simulink model "impmodel"  (R2023a)
settings: Solver=FixedStepDiscrete  StartTime=0.0  StopTime=8  RelTol=1e-3  EnableMultiTasking=on
values from neighbouring files (symbols this model uses):
  availableSpeedModes = 3    [params_f2838.mat]
  inverter_DRV8300 =     [params_f2838.mat]
  PI_params =     [params_f2838.mat]
  pmsm_ECI6360 =     [params_f2838.mat]
  PU_System =     [params_f2838.mat]
  target_f2838 =     [params_f2838.mat]
  Ts = 5e-05    [params_f2838.mat]
  Ts_motor = 2.5e-05    [params_f2838.mat]
  Ts_simulink = 2.5e-05    [params_f2838.mat]
  Ts_speed = 0.0005    [params_f2838.mat]
undefined symbols (not defined in the file or in its folder): Down, GPTRIP1SEL, TZ1, Up
libraries: simulink x35, c2802xlib x11, idelinklib_common x8, procinterlib x8, mcbcontrolslib x8, c280xlib x7, mcbpositiondecoderlib x7, slpidlib x5, svdschedulerlib x4, c2838xlib x2, autolibpmsminterior x1, mcbplantlib x1
(part 1 of 4)
settings Model: ExtModeTrigDuration=8  Creator=baris  LastModifiedBy=baris
settings SolverCC: AutoInsertRateTranBlk=on
settings DataIOCC: LimitDataPoints=on  SaveFormat=Array  SaveOutput=off  SaveTime=off  ReturnWorkspaceOutputs=off
settings OptimizationCC: DefaultUnderspecifiedDataType=single  EnhancedBackFolding=on  PassReuseOutputArgsAs=Individual arguments  MaxStackSize=1024  OptimizeBlockOrder=speed  DifferentSizesBufferReuse=on  DenormalBehavior=FlushToZero  EfficientTunableParamExpr=on
settings DebuggingCC: ReadBeforeWriteMsg=DisableAll  WriteAfterWriteMsg=DisableAll  WriteAfterReadMsg=DisableAll  SignalResolutionControl=TryResolveAllWithWarning  InheritedTsInSrcMsg=none  MultiTaskDSMMsg=none  MultiTaskCondExecSysMsg=none  TasksWithSamePriorityMsg=none  SigSpecEnsureSampleTimeMsg=none  IntegerOverflowMsg=none  ParameterPrecisionLossMsg=none  FcnCallInpInsideContextMsg=warning  UnconnectedInputMsg=warning  UnconnectedOutputMsg=warning  UnconnectedLineMsg=warning  IntegerSaturationMsg=none
settings HardwareCC: ProdBitPerChar=16  ProdBitPerInt=16  ProdBitPerPointer=32  ProdBitPerSizeT=32  ProdBitPerPtrDiffT=32  ProdLargestAtomicInteger=Integer  ProdLargestAtomicFloat=None  ProdWordSize=16  ProdLongLongMode=on  ProdHWDeviceType=Texas Instruments->C2000  HardwareBoardFeatureSet=SoCBlockset
settings ModelReferenceCC: EnableRefExpFcnMdlSchedulingChecks=on  PropagateSignalLabelsOutOfModel=off
settings SFSimCC: MATLABDynamicMemAlloc=off
settings RTWCC: Description=Embedded Coder  SystemTargetFile=ert.tlc  HardwareBoard=TI F2838x  TemplateMakefile=ert_default_tmf  CustomDefine=-DCARPEDIEM_PIN_CORRECTION  Toolchain=Texas Instruments Code Composer Studio - EABI (C2000)
settings CodeAppCC: ForceParamTrailComments=on  IgnoreCustomStorageClasses=off  OperatorAnnotations=on  SimulinkDataObjDesc=on  SFDataObjDesc=on  InsertBlockDesc=on
settings ERTTargetCC: CodeReplacementLibrary=TI C28x  ExtModeTransport=4  ExtModeStaticAlloc=on  ExtModeAutomaticAllocSize=off  ExtModeStaticAllocSize=10000  ExtModeMexFile=ext_xcp  ExtModeIntrfLevel=Level2 - Open
settings ConfigComp: CovEnable=on  RecordCoverage=on  CovModelRefEnable=on

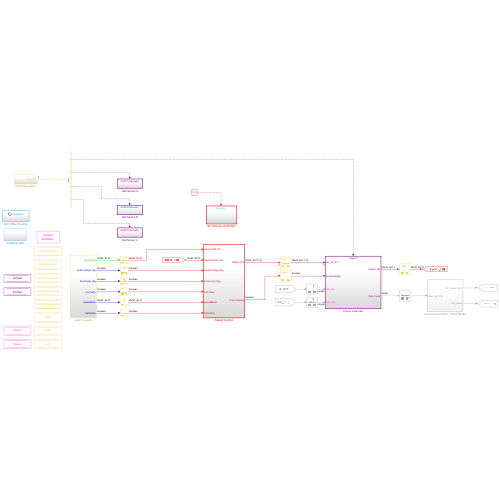
[thumbnail: Simulink's stored preview of the top-level diagram]
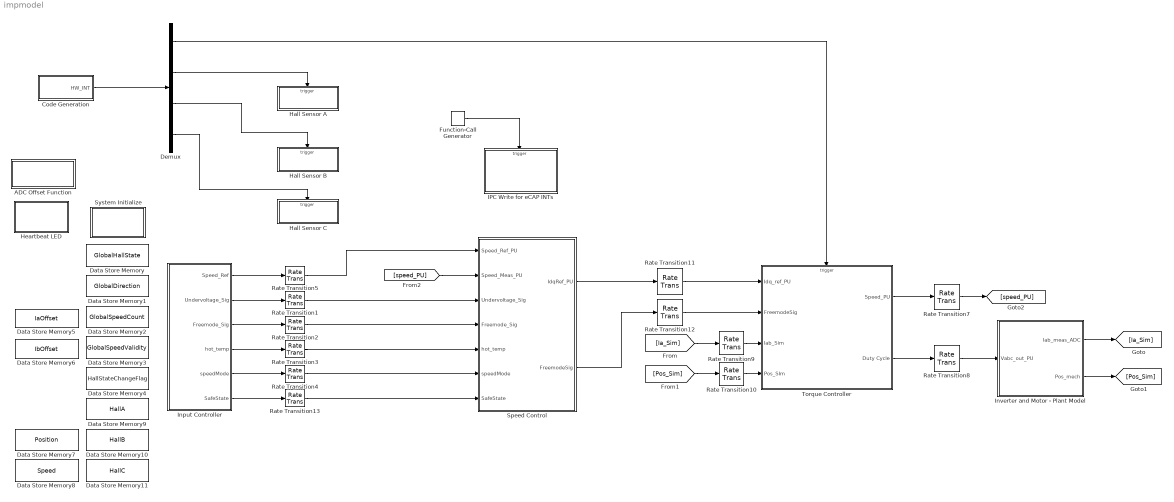
== system impmodel ==
  ADC Offset Function : Subsystem  TreatAsAtomicUnit=on
  Code Generation : Subsystem
  Data Store Memory : DataStoreMemory  DataStoreName=GlobalHallState  WriteAfterWriteMsg=warning  ShowAdditionalParam=off
  Data Store Memory1 : DataStoreMemory  DataStoreName=GlobalDirection  WriteAfterWriteMsg=warning  ShowAdditionalParam=off
  Data Store Memory10 : DataStoreMemory  DataStoreName=HallB  WriteAfterWriteMsg=warning  ShowAdditionalParam=off
  Data Store Memory11 : DataStoreMemory  DataStoreName=HallC  WriteAfterWriteMsg=warning  ShowAdditionalParam=off
  Data Store Memory2 : DataStoreMemory  DataStoreName=GlobalSpeedCount  WriteAfterWriteMsg=warning  ShowAdditionalParam=off
  Data Store Memory3 : DataStoreMemory  DataStoreName=GlobalSpeedValidity  WriteAfterWriteMsg=warning  ShowAdditionalParam=off
  Data Store Memory4 : DataStoreMemory  DataStoreName=HallStateChangeFlag  WriteAfterWriteMsg=warning  ShowAdditionalParam=off
  Data Store Memory5 : DataStoreMemory  DataStoreName=IaOffset  WriteAfterWriteMsg=warning  ShowAdditionalParam=off
  Data Store Memory6 : DataStoreMemory  DataStoreName=IbOffset  WriteAfterWriteMsg=warning  ShowAdditionalParam=off
  Data Store Memory7 : DataStoreMemory  DataStoreName=Position  WriteAfterWriteMsg=warning  ShowAdditionalParam=off
  Data Store Memory8 : DataStoreMemory  DataStoreName=Speed  WriteAfterWriteMsg=warning  ShowAdditionalParam=off
  Data Store Memory9 : DataStoreMemory  DataStoreName=HallA  WriteAfterWriteMsg=warning  ShowAdditionalParam=off
  Demux : Demux
  Function-Call Generator : simulink/Ports & Subsystems/Function-Call Generator  sample_time=-1  numberOfIterations=1  DisallowWideOutput=off
  Hall Sensor A : Subsystem
  Hall Sensor B : Subsystem
  Hall Sensor C : Subsystem
  Heartbeat LED : Subsystem
  IPC Write for eCAP INTs : Subsystem
  Input Controller : Subsystem
  Inverter and Motor - Plant Model : Subsystem
  Rate Transition1 : RateTransition  Deterministic=off  OutPortSampleTime=Ts_speed
  Rate Transition{9..12} (4 alike) : RateTransition  Deterministic=off
  Rate Transition{2..4,13} (4 alike) : RateTransition  Integrity=off  Deterministic=off  OutPortSampleTime=Ts_speed
  Rate Transition5 : RateTransition  Deterministic=off  OutPortSampleTime=Ts_speed
  Rate Transition7 : RateTransition  Deterministic=off  OutPortSampleTime=Ts_speed
  Rate Transition8 : RateTransition  Deterministic=off  OutPortSampleTime=Ts_simulink
  Speed Control : Subsystem  TreatAsAtomicUnit=on  SystemSampleTime=Ts_speed
  System Initialize : Subsystem  mask(System Initialize){ShowInLibBrowser=0}
      mask prompts: ShowInLibBrowser "Simulink:masks:CustCodeMaskParam1_MP"
      settings: CopyFcn=cccopyfcn(gcb)  OpenFcn=ccopenfcn('System Initialize Function')
      mask Help: eval('feval(''rtwprivate'',''rtwhelpview'',''rtw_sys_initialize_block'')');
      mask DialogControl ShowInLibBrowser Prompt: Mask Parameter 1:
      mask Display: disp('System\nInitialize');
  Torque Controller : Subsystem
  wires:
  Code Generation/1(HW_INT) -> Demux/1
  Demux/1 -> Torque Controller/Trigger
  Rate Transition5/1 -> Speed Control/1(Speed_Ref_PU)
  Torque Controller/1(Speed_PU) -> Rate Transition7/1
  [speed_PU] -> Speed Control/2(Speed_Meas_PU)
  Input Controller/1(Speed_Ref) -> Rate Transition5/1
  Input Controller/2(Undervoltage_Sig) -> Rate Transition1/1
  Input Controller/3(Freemode_Sig) -> Rate Transition2/1
  Input Controller/4(hot_temp) -> Rate Transition3/1
  Input Controller/5(speedMode) -> Rate Transition4/1
  Rate Transition1/1 -> Speed Control/3(Undervoltage_Sig)
  Rate Transition2/1 -> Speed Control/4(Freemode_Sig)
  Rate Transition3/1 -> Speed Control/5(hot_temp)
  Rate Transition4/1 -> Speed Control/6(speedMode)
  Inverter and Motor - Plant Model/1(Iab_meas_ADC) -> [Ia_Sim]
  Inverter and Motor - Plant Model/2(Pos_mech) -> [Pos_Sim]
  Torque Controller/2(Duty Cycle) -> Rate Transition8/1
  Rate Transition8/1 -> Inverter and Motor - Plant Model/1(Vabc_out_PU)
  Rate Transition10/1 -> Torque Controller/4(Pos_SIm)
  [Pos_Sim] -> Rate Transition10/1
  [Ia_Sim] -> Rate Transition9/1
  Rate Transition9/1 -> Torque Controller/3(Iab_Sim)
  Speed Control/1(IdqRef_PU) -> Rate Transition11/1
  Speed Control/2(FreemodeSig) -> Rate Transition12/1
  Rate Transition11/1 -> Torque Controller/1(Idq_ref_PU)
  Rate Transition12/1 -> Torque Controller/2(FreemodeSig)
  Rate Transition7/1 -> [speed_PU]
  Input Controller/6(SafeState) -> Rate Transition13/1
  Rate Transition13/1 -> Speed Control/7(SafeState)
  Demux/2 -> Hall Sensor A/Trigger
  Demux/3 -> Hall Sensor B/Trigger
  Demux/4 -> Hall Sensor C/Trigger
  Function-Call Generator/1 -> IPC Write for eCAP INTs/Trigger

== system impmodel/ADC Offset Function ==
  "Calculate ADC Offset " : Subsystem  Priority=1001  TreatAsAtomicUnit=on
  Constant : Constant  Value=inverter_DRV8300.ADCOffsetCalibEnable
  Default ADC Offset : Subsystem  Priority=1001  TreatAsAtomicUnit=on
  Event Listener : EventListener  DisableCoverage=on  EventName=reset
  NOT : Logic  Operator=NOT  IconShape=distinctive  AllPortsSameDT=off  OutDataTypeStr=boolean
  wires:
  Constant/1 -> NOT/1, "Calculate ADC Offset "/Enable
  NOT/1 -> Default ADC Offset/Enable

== system impmodel/Code Generation ==
  CodeGeneration : Subsystem
  Simulation : Subsystem
  Variant Source : VariantSource  VariantControlMode=sim codegen switching  OutputFunctionCall=on
  HW_INT : Outport
  wires:
  Variant Source/1 -> HW_INT/1
  CodeGeneration/1(HW_INT) -> Variant Source/1
  Simulation/1(HW_INT) -> Variant Source/2

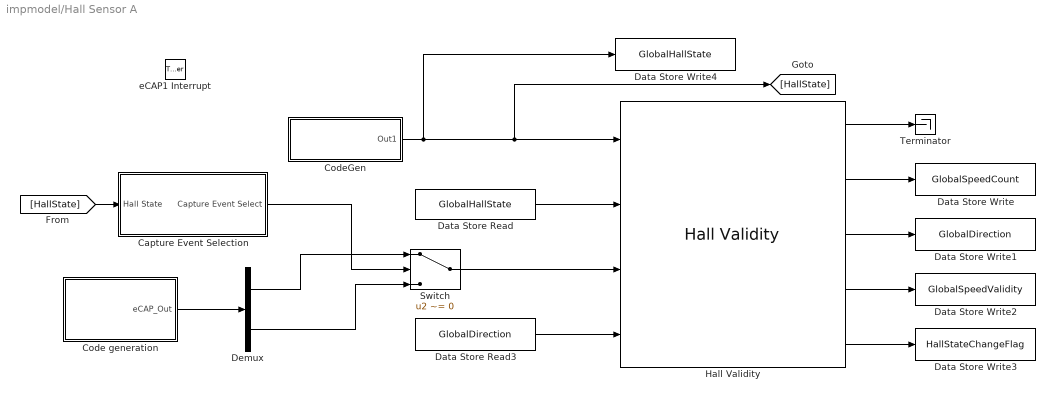
== system impmodel/Hall Sensor A ==
  eCAP1 Interrupt : TriggerPort  TriggerType=function-call  VariantControl=(inherit)  PortDimensions=1
  Capture Event Selection : Subsystem
  Code generation : Subsystem
  CodeGen : Subsystem
  Data Store Read : DataStoreRead  DataStoreName=GlobalHallState  IndexOptions=Index vector (dialog)  Indices=1  OutputSizes=1
  Data Store Read3 : DataStoreRead  DataStoreName=GlobalDirection  IndexOptions=Index vector (dialog)  Indices=1  OutputSizes=1
  Data Store Write : DataStoreWrite  DataStoreName=GlobalSpeedCount  IndexOptions=Index vector (dialog)  Indices=1  OutputSizes=1
  Data Store Write1 : DataStoreWrite  DataStoreName=GlobalDirection  IndexOptions=Index vector (dialog)  Indices=1  OutputSizes=1
  Data Store Write2 : DataStoreWrite  DataStoreName=GlobalSpeedValidity  IndexOptions=Index vector (dialog)  Indices=1  OutputSizes=1
  Data Store Write3 : DataStoreWrite  DataStoreName=HallStateChangeFlag  IndexOptions=Index vector (dialog)  Indices=1  OutputSizes=1
  Data Store Write4 : DataStoreWrite  DataStoreName=GlobalHallState  IndexOptions=Index vector (dialog)  Indices=1  OutputSizes=1
  Demux : Demux  Outputs=2
  Hall Validity : mcbpositiondecoderlib/Hall Validity  hallSequence=ABC  sequence=[5,4,6,2,3,1]  CounterSize=32 bits
      settings: LibrarySourceBlock=mcblib/Sensor Decoders/Hall Validity
  Switch : Switch  Criteria=u2 ~= 0  SaturateOnIntegerOverflow=off  InputSameDT=off
  Terminator : Terminator
  wires:
  Hall Validity/4 -> Data Store Write2/1
  Hall Validity/1 -> Terminator/1
  Hall Validity/5 -> Data Store Write3/1
  Data Store Read3/1 -> Hall Validity/4
  CodeGen/1(Out1) -> Hall Validity/1, [HallState], Data Store Write4/1
  Hall Validity/2 -> Data Store Write/1
  Hall Validity/3 -> Data Store Write1/1
  [HallState] -> Capture Event Selection/1(Hall State)
  Switch/1 -> Hall Validity/3
  Capture Event Selection/1(Capture Event Select) -> Switch/2
  Code generation/1(eCAP_Out) -> Demux/1
  Data Store Read/1 -> Hall Validity/2
  Demux/1 -> Switch/1
  Demux/2 -> Switch/3

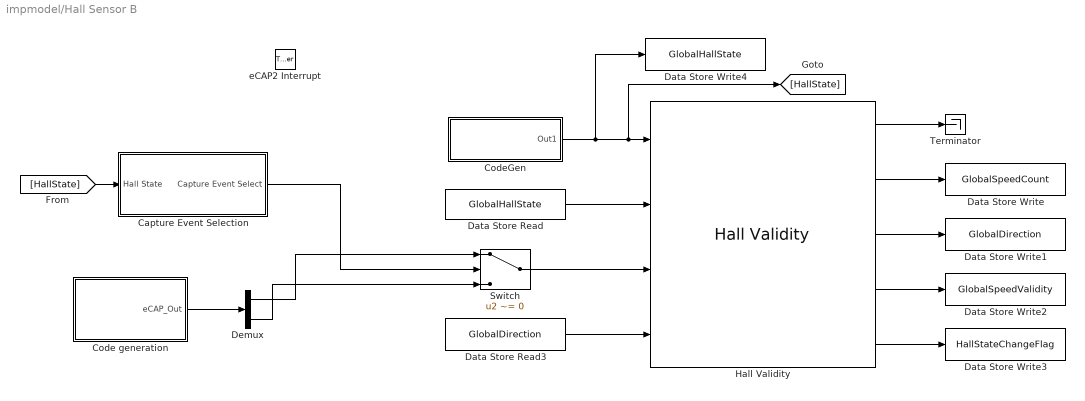
== system impmodel/Hall Sensor B ==
  eCAP2 Interrupt : TriggerPort  TriggerType=function-call  VariantControl=(inherit)  PortDimensions=1
  Capture Event Selection : Subsystem
  Code generation : Subsystem
  CodeGen : Subsystem
  Data Store Read : DataStoreRead  DataStoreName=GlobalHallState  IndexOptions=Index vector (dialog)  Indices=1  OutputSizes=1
  Data Store Read3 : DataStoreRead  DataStoreName=GlobalDirection  IndexOptions=Index vector (dialog)  Indices=1  OutputSizes=1
  Data Store Write : DataStoreWrite  DataStoreName=GlobalSpeedCount  IndexOptions=Index vector (dialog)  Indices=1  OutputSizes=1
  Data Store Write1 : DataStoreWrite  DataStoreName=GlobalDirection  IndexOptions=Index vector (dialog)  Indices=1  OutputSizes=1
  Data Store Write2 : DataStoreWrite  DataStoreName=GlobalSpeedValidity  IndexOptions=Index vector (dialog)  Indices=1  OutputSizes=1
  Data Store Write3 : DataStoreWrite  DataStoreName=HallStateChangeFlag  IndexOptions=Index vector (dialog)  Indices=1  OutputSizes=1
  Data Store Write4 : DataStoreWrite  DataStoreName=GlobalHallState  IndexOptions=Index vector (dialog)  Indices=1  OutputSizes=1
  Demux : Demux  Outputs=2
  Hall Validity : mcbpositiondecoderlib/Hall Validity  hallSequence=ABC  sequence=[5,4,6,2,3,1]  CounterSize=32 bits
      settings: LibrarySourceBlock=mcblib/Sensor Decoders/Hall Validity
  Switch : Switch  Criteria=u2 ~= 0  SaturateOnIntegerOverflow=off  InputSameDT=off
  Terminator : Terminator
  wires:
  Hall Validity/3 -> Data Store Write1/1
  Hall Validity/2 -> Data Store Write/1
  CodeGen/1(Out1) -> [HallState], Hall Validity/1, Data Store Write4/1
  Data Store Read3/1 -> Hall Validity/4
  Hall Validity/5 -> Data Store Write3/1
  Hall Validity/1 -> Terminator/1
  Hall Validity/4 -> Data Store Write2/1
  Capture Event Selection/1(Capture Event Select) -> Switch/2
  [HallState] -> Capture Event Selection/1(Hall State)
  Code generation/1(eCAP_Out) -> Demux/1
  Demux/1 -> Switch/1
  Demux/2 -> Switch/3
  Switch/1 -> Hall Validity/3
  Data Store Read/1 -> Hall Validity/2

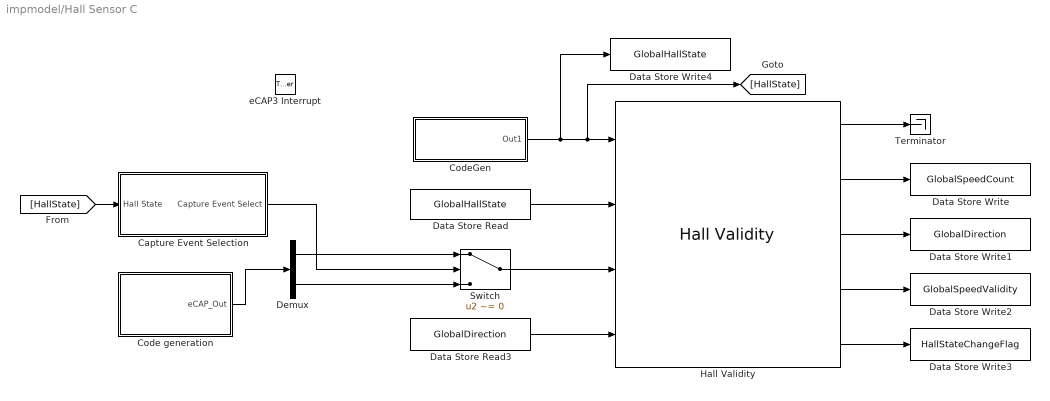
== system impmodel/Hall Sensor C ==
  eCAP3 Interrupt : TriggerPort  TriggerType=function-call  VariantControl=(inherit)  PortDimensions=1
  Capture Event Selection : Subsystem
  Code generation : Subsystem
  CodeGen : Subsystem
  Data Store Read : DataStoreRead  DataStoreName=GlobalHallState  IndexOptions=Index vector (dialog)  Indices=1  OutputSizes=1
  Data Store Read3 : DataStoreRead  DataStoreName=GlobalDirection  IndexOptions=Index vector (dialog)  Indices=1  OutputSizes=1
  Data Store Write : DataStoreWrite  DataStoreName=GlobalSpeedCount  IndexOptions=Index vector (dialog)  Indices=1  OutputSizes=1
  Data Store Write1 : DataStoreWrite  DataStoreName=GlobalDirection  IndexOptions=Index vector (dialog)  Indices=1  OutputSizes=1
  Data Store Write2 : DataStoreWrite  DataStoreName=GlobalSpeedValidity  IndexOptions=Index vector (dialog)  Indices=1  OutputSizes=1
  Data Store Write3 : DataStoreWrite  DataStoreName=HallStateChangeFlag  IndexOptions=Index vector (dialog)  Indices=1  OutputSizes=1
  Data Store Write4 : DataStoreWrite  DataStoreName=GlobalHallState  IndexOptions=Index vector (dialog)  Indices=1  OutputSizes=1
  Demux : Demux  Outputs=2
  Hall Validity : mcbpositiondecoderlib/Hall Validity  hallSequence=ABC  sequence=[5,4,6,2,3,1]  CounterSize=32 bits
      settings: LibrarySourceBlock=mcblib/Sensor Decoders/Hall Validity
  Switch : Switch  Criteria=u2 ~= 0  SaturateOnIntegerOverflow=off  InputSameDT=off
  Terminator : Terminator
  wires:
  Hall Validity/4 -> Data Store Write2/1
  Hall Validity/1 -> Terminator/1
  Hall Validity/5 -> Data Store Write3/1
  Data Store Read3/1 -> Hall Validity/4
  CodeGen/1(Out1) -> Data Store Write4/1, [HallState], Hall Validity/1
  Hall Validity/2 -> Data Store Write/1
  Hall Validity/3 -> Data Store Write1/1
  [HallState] -> Capture Event Selection/1(Hall State)
  Switch/1 -> Hall Validity/3
  Code generation/1(eCAP_Out) -> Demux/1
  Demux/1 -> Switch/1
  Demux/2 -> Switch/3
  Capture Event Selection/1(Capture Event Select) -> Switch/2
  Data Store Read/1 -> Hall Validity/2

== system impmodel/Heartbeat LED ==
  Constant : Constant  SampleTime=0.5
  Digital Output : c2838xlib/Digital Output  GPIO_Number=GPIO56~GPIO63  GPIO_Bit0=on  GPIO_BIT0_Toggle=on  GPIO_Bit1=off  GPIO_BIT1_Toggle=off  GPIO_Bit2=off  GPIO_BIT2_Toggle=off  GPIO_Bit3=off  GPIO_BIT3_Toggle=off  GPIO_Bit4=off  GPIO_BIT4_Toggle=off  GPIO_Bit5=off  GPIO_BIT5_Toggle=off  GPIO_Bit6=off  GPIO_BIT6_Toggle=off  GPIO_Bit7=off  GPIO_BIT7_Toggle=off
  wires:
  Constant/1 -> Digital Output/1

== system impmodel/IPC Write for eCAP INTs ==
  function : TriggerPort  TriggerType=function-call  VariantControl=(inherit)
  Data Store Read2 : DataStoreRead  DataStoreName=GlobalHallState  IndexOptions=Index vector (dialog)  Indices=1  OutputSizes=1
  Data Store Read3 : DataStoreRead  DataStoreName=HallA  IndexOptions=Index vector (dialog)  Indices=1  OutputSizes=1
  Data Store Read4 : DataStoreRead  DataStoreName=HallB  IndexOptions=Index vector (dialog)  Indices=1  OutputSizes=1
  Data Store Read5 : DataStoreRead  DataStoreName=HallC  IndexOptions=Index vector (dialog)  Indices=1  OutputSizes=1
  Memory{2..5} (4 alike) : Memory  InheritSampleTime=on
  TCP_HallA : Subsystem
  TCP_HallB : Subsystem
  TCP_HallC : Subsystem
  TCP_HallState : Subsystem
  wires:
  Data Store Read2/1 -> Memory2/1
  Data Store Read3/1 -> Memory3/1
  Data Store Read4/1 -> Memory4/1
  Data Store Read5/1 -> Memory5/1
  Memory2/1 -> TCP_HallState/1(" ")
  Memory3/1 -> TCP_HallA/1(" ")
  Memory4/1 -> TCP_HallB/1(" ")
  Memory5/1 -> TCP_HallC/1(" ")

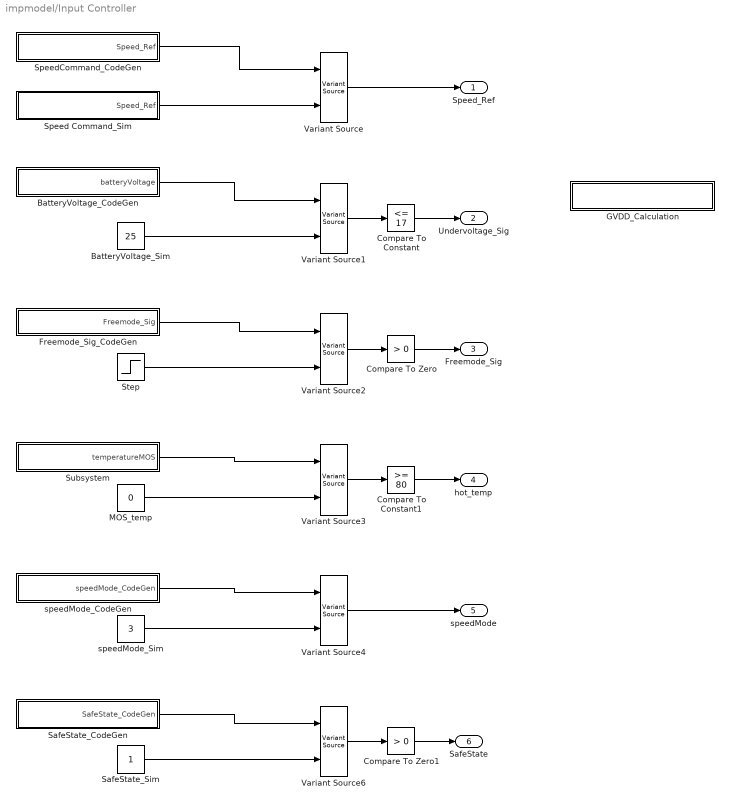
== system impmodel/Input Controller ==
  BatteryVoltage_CodeGen : Subsystem
  BatteryVoltage_Sim : Constant  Value=25  OutDataTypeStr=uint16  SampleTime=0.2
  Compare To Constant : simulink/Logic and Bit Operations/Compare To Constant  relop=<=  const=17  OutDataTypeStr=boolean
  Compare To Constant1 : simulink/Logic and Bit Operations/Compare To Constant  relop=>=  const=80  OutDataTypeStr=boolean
  Compare To Zero : simulink/Logic and Bit Operations/Compare To Zero  relop=>  OutDataTypeStr=boolean
  Compare To Zero1 : simulink/Logic and Bit Operations/Compare To Zero  relop=>  OutDataTypeStr=boolean
  Freemode_Sig_CodeGen : Subsystem
  GVDD_Calculation : Subsystem
  MOS_temp : Constant  Value=0  OutDataTypeStr=uint16  SampleTime=0.2
  SafeState_CodeGen : Subsystem
  SafeState_Sim : Constant  OutDataTypeStr=uint8  SampleTime=0.2
  Speed Command_Sim : Subsystem
  SpeedCommand_CodeGen : Subsystem
  Step : Step  Time=10  After=0  SampleTime=0.2
  Subsystem : Subsystem
  Variant Source{,1..4,6} (6 alike) : VariantSource  VariantControlMode=sim codegen switching
  speedMode_CodeGen : Subsystem
  speedMode_Sim : Constant  Value=3  OutDataTypeStr=uint16  SampleTime=0.2
  Speed_Ref : Outport
  Undervoltage_Sig : Outport  Port=2
  Freemode_Sig : Outport  Port=3
  hot_temp : Outport  Port=4
  speedMode : Outport  Port=5
  SafeState : Outport  Port=6
  wires:
  Variant Source/1 -> Speed_Ref/1
  SpeedCommand_CodeGen/1(Speed_Ref) -> Variant Source/1
  Speed Command_Sim/1(Speed_Ref) -> Variant Source/2
  Variant Source1/1 -> Compare To Constant/1
  BatteryVoltage_CodeGen/1(batteryVoltage) -> Variant Source1/1
  BatteryVoltage_Sim/1 -> Variant Source1/2
  Compare To Constant/1 -> Undervoltage_Sig/1
  Variant Source2/1 -> Compare To Zero/1
  Step/1 -> Variant Source2/2
  Freemode_Sig_CodeGen/1(Freemode_Sig) -> Variant Source2/1
  Subsystem/1(temperatureMOS) -> Variant Source3/1
  MOS_temp/1 -> Variant Source3/2
  Variant Source3/1 -> Compare To Constant1/1
  Compare To Constant1/1 -> hot_temp/1
  Variant Source4/1 -> speedMode/1
  speedMode_Sim/1 -> Variant Source4/2
  speedMode_CodeGen/1(speedMode_CodeGen) -> Variant Source4/1
  Compare To Zero/1 -> Freemode_Sig/1
  Variant Source6/1 -> Compare To Zero1/1
  SafeState_Sim/1 -> Variant Source6/2
  SafeState_CodeGen/1(SafeState_CodeGen) -> Variant Source6/1
  Compare To Zero1/1 -> SafeState/1

== system impmodel/Inverter and Motor - Plant Model ==
  Vabc_out_PU : Inport
  Codegeneration : Subsystem
  Simulation : Subsystem
  Variant Sink : VariantSink  VariantControlMode=sim codegen switching
  Variant Source : VariantSource  VariantControlMode=sim codegen switching
  Variant Source1 : VariantSource  VariantControlMode=sim codegen switching
  Iab_meas_ADC : Outport  VectorParamsAs1DForOutWhenUnconnected=off
  Pos_mech : Outport  Port=2  VectorParamsAs1DForOutWhenUnconnected=off
  wires:
  Codegeneration/2(Pos_fb_Sim) -> Variant Source1/1
  Codegeneration/1(Iab_fb_Sim) -> Variant Source/1
  Variant Source1/1 -> Pos_mech/1
  Variant Sink/1 -> Codegeneration/1(Duty_Cycles)
  Variant Source/1 -> Iab_meas_ADC/1
  Simulation/1(Iab_fb_Sim) -> Variant Source/2
  Variant Sink/2 -> Simulation/1(Duty_Cycles)
  Simulation/2(Pos_fb_Sim) -> Variant Source1/2
  Vabc_out_PU/1 -> Variant Sink/1

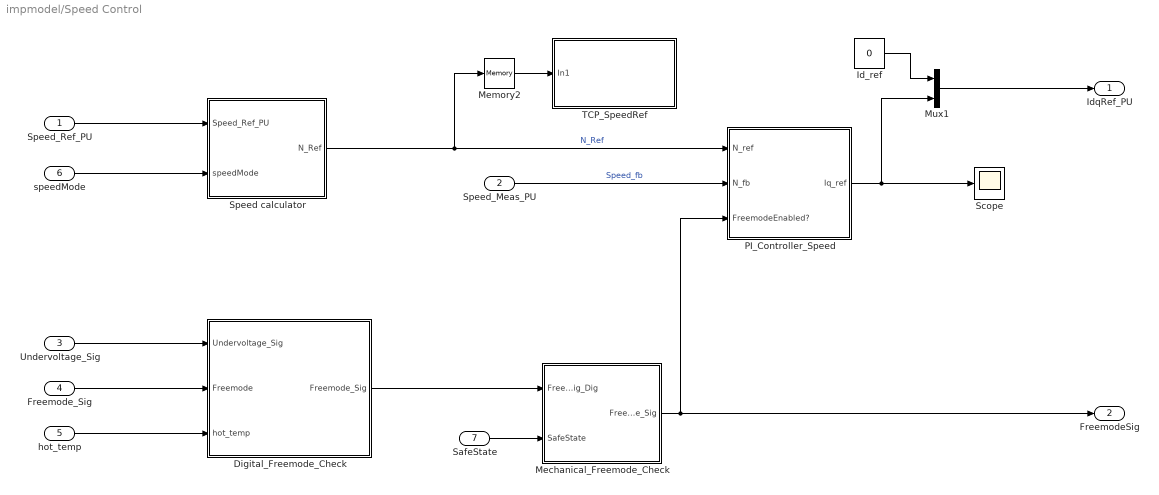
== system impmodel/Speed Control ==
  Speed_Ref_PU : Inport
  Speed_Meas_PU : Inport  Port=2
  Undervoltage_Sig : Inport  Port=3
  Freemode_Sig : Inport  Port=4
  hot_temp : Inport  Port=5
  speedMode : Inport  Port=6
  SafeState : Inport  Port=7
  Digital_Freemode_Check : Subsystem  TreatAsAtomicUnit=on
  Id_ref : Constant  Value=0  OutDataTypeStr=fixdt(1,32,17)  SampleTime=Ts_speed
  Mechanical_Freemode_Check : Subsystem
  Memory2 : Memory  InheritSampleTime=on
  Mux1 : Mux  Inputs=2
  PI_Controller_Speed : Subsystem  TreatAsAtomicUnit=on  SystemSampleTime=Ts_speed
  Scope : Scope
  Speed calculator : Subsystem
  TCP_SpeedRef : Subsystem
  IdqRef_PU : Outport  VectorParamsAs1DForOutWhenUnconnected=off
  FreemodeSig : Outport  Port=2  VectorParamsAs1DForOutWhenUnconnected=off
  wires:
  Id_ref/1 -> Mux1/1
  speedMode/1 -> Speed calculator/2(speedMode)
  Freemode_Sig/1 -> Digital_Freemode_Check/2(Freemode)
  Undervoltage_Sig/1 -> Digital_Freemode_Check/1(Undervoltage_Sig)
  hot_temp/1 -> Digital_Freemode_Check/3(hot_temp)
  Speed_Meas_PU/1 -> PI_Controller_Speed/2(N_fb)  "Speed_fb"
  Mux1/1 -> IdqRef_PU/1
  Speed calculator/1(N_Ref) -> Memory2/1, PI_Controller_Speed/1(N_ref)  "N_Ref"
  Speed_Ref_PU/1 -> Speed calculator/1(Speed_Ref_PU)
  SafeState/1 -> Mechanical_Freemode_Check/2(SafeState)
  PI_Controller_Speed/1(Iq_ref) -> Scope/1, Mux1/2
  Digital_Freemode_Check/1("Freemode_Sig  ") -> Mechanical_Freemode_Check/1(Freemode_Sig_Dig)
  Mechanical_Freemode_Check/1(Freemode_Sig) -> PI_Controller_Speed/3("  FreemodeEnabled?"), FreemodeSig/1
  Memory2/1 -> TCP_SpeedRef/1(In1)

== system impmodel/System Initialize ==

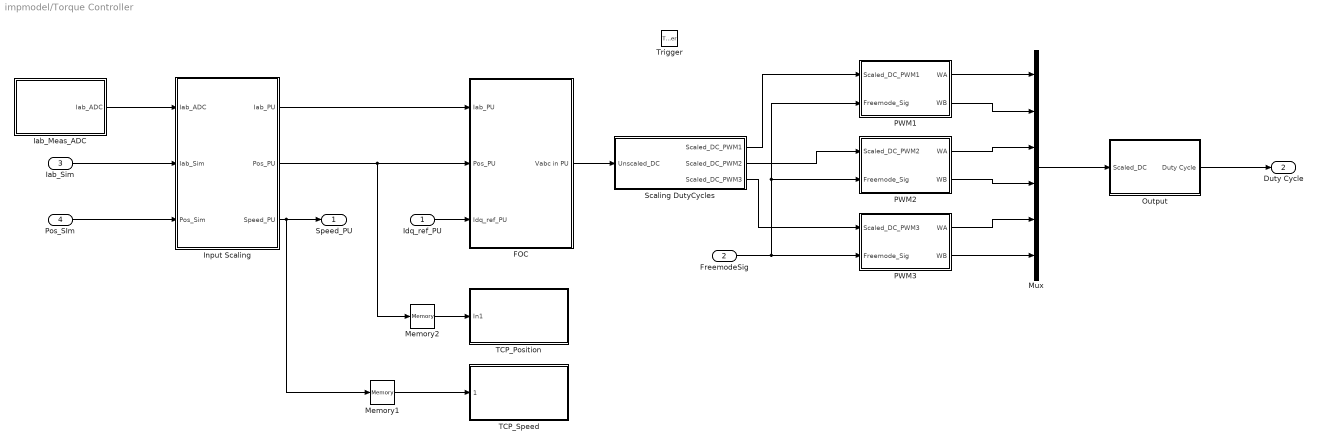
== system impmodel/Torque Controller ==
  Idq_ref_PU : Inport
  FreemodeSig : Inport  Port=2
  Iab_Sim : Inport  Port=3
  Pos_SIm : Inport  Port=4
  Trigger : TriggerPort  TriggerType=function-call  VariantControl=(inherit)  PortDimensions=1
  FOC : Subsystem
  Iab_Meas_ADC : Subsystem
  Input Scaling : Subsystem
  Memory1 : Memory  InheritSampleTime=on
  Memory2 : Memory  InheritSampleTime=on
  Mux : Mux  Inputs=6
  Output : Subsystem
  PWM1 : Subsystem
  PWM2 : Subsystem
  PWM3 : Subsystem
  Scaling DutyCycles : Subsystem
  TCP_Position : Subsystem
  TCP_Speed : Subsystem
  Speed_PU : Outport
  Duty Cycle : Outport  Port=2
  wires:
  Input Scaling/3(Speed_PU) -> Memory1/1, Speed_PU/1
  Idq_ref_PU/1 -> FOC/3(Idq_ref_PU)
  Iab_Meas_ADC/1(Iab_ADC) -> Input Scaling/1(Iab_ADC)
  Iab_Sim/1 -> Input Scaling/2(Iab_Sim)
  Pos_SIm/1 -> Input Scaling/3(Pos_Sim)
  PWM1/2(WB) -> Mux/2
  PWM3/2(WB) -> Mux/6
  Scaling DutyCycles/2(Scaled_DC_PWM2) -> PWM2/1(Scaled_DC_PWM2)
  PWM2/1(WA) -> Mux/3
  Scaling DutyCycles/3(Scaled_DC_PWM3) -> PWM3/1(Scaled_DC_PWM3)
  PWM1/1(WA) -> Mux/1
  Scaling DutyCycles/1(Scaled_DC_PWM1) -> PWM1/1(Scaled_DC_PWM1)
  PWM2/2(WB) -> Mux/4
  PWM3/1(WA) -> Mux/5
  FreemodeSig/1 -> PWM3/2(Freemode_Sig), PWM1/2(Freemode_Sig), PWM2/2(Freemode_Sig)
  FOC/1(Vabc in PU) -> Scaling DutyCycles/1(Unscaled_DC)
  Output/1(Duty Cycle) -> Duty Cycle/1
  Mux/1 -> Output/1(Scaled_DC)
  Input Scaling/1(Iab_PU) -> FOC/1(Iab_PU)
  Input Scaling/2(Pos_PU) -> Memory2/1, FOC/2(Pos_PU)
  Memory1/1 -> TCP_Speed/1(" ")
  Memory2/1 -> TCP_Position/1(In1)

== system impmodel/ADC Offset Function/Calculate ADC Offset  ==
  Enable : EnablePort
  Constant : Constant  Value=8
  Constant1 : Constant  Value=inverter_DRV8300.CtSensOffsetMax  OutDataTypeStr=Inherit: Inherit via back propagation
  Constant2 : Constant  Value=inverter_DRV8300.CtSensOffsetMin  OutDataTypeStr=Inherit: Inherit via back propagation
  Divide : Product  Inputs=*/  OutDataTypeStr=uint16
  Divide1 : Product  Inputs=*/  OutDataTypeStr=uint16
  For Iterator Subsystem : Subsystem  TreatAsAtomicUnit=on
  If : If  NumInputs=3  IfExpression=u1 > u3 & u1 < u2
  If Action Subsystem : Subsystem  TreatAsAtomicUnit=on
  If Action Subsystem1 : Subsystem  TreatAsAtomicUnit=on
  If Action Subsystem2 : Subsystem  TreatAsAtomicUnit=on
  If Action Subsystem3 : Subsystem  TreatAsAtomicUnit=on
  If1 : If  NumInputs=3  IfExpression=u1 > u3 & u1 < u2
  wires:
  For Iterator Subsystem/1(Out1) -> Divide/1
  If1/2 -> If Action Subsystem3/Action
  If1/1 -> If Action Subsystem2/Action
  If/2 -> If Action Subsystem1/Action
  For Iterator Subsystem/2(Out2) -> Divide1/1
  If/1 -> If Action Subsystem/Action
  Constant2/1 -> If/3, If1/3
  Constant1/1 -> If/2, If1/2
  Divide1/1 -> If1/1, If Action Subsystem2/1(In1)
  Constant/1 -> Divide/2, Divide1/2
  Divide/1 -> If Action Subsystem/1(In1), If/1

== system impmodel/ADC Offset Function/Default ADC Offset ==
  Enable : EnablePort
  Constant : Constant  Value=inverter_DRV8300.CtSensAOffset  OutDataTypeStr=Inherit: Inherit via back propagation
  Constant1 : Constant  Value=inverter_DRV8300.CtSensBOffset  OutDataTypeStr=Inherit: Inherit via back propagation
  Data Store Write1 : DataStoreWrite  DataStoreName=IaOffset  IndexOptions=Index vector (dialog)  Indices=1  OutputSizes=1
  Data Store Write2 : DataStoreWrite  DataStoreName=IbOffset  IndexOptions=Index vector (dialog)  Indices=1  OutputSizes=1
  wires:
  Constant/1 -> Data Store Write1/1
  Constant1/1 -> Data Store Write2/1

== system impmodel/Code Generation/CodeGeneration ==
  HW_INT_ADCB1 : svdschedulerlib/Hardware Interrupt v2  ISRGroup=ADC - Analog to Digital Converter  ISRName=ADCA1_INT  ISRNumber=32  NumEventsToServe=1  EventsList={'on','EOC event','1';'off','Overflow event','2';'off','Custom event','3'}  SelectedEvents={'event1'}  TaskPriority=30  DisablePreemption=off  ClearInterruptFlagsAtEndOfEvent=on  InterruptDefinitionFile=$(TARGET_ROOT)/registry/interrupts/F2837xS_interrupts.xml  HardwareBoard=F2837x  EnableSimPort=off
      settings: LibrarySourceBlock=c2000lib/Scheduling/Hardware Interrupt
  HW_INT_ECAP1 : svdschedulerlib/Hardware Interrupt v2  ISRGroup=ADC - Analog to Digital Converter  ISRName=ADCA1_INT  ISRNumber=32  NumEventsToServe=1  EventsList={'on','EOC event','1';'off','Overflow event','2';'off','Custom event','3'}  SelectedEvents={'event1'}  TaskPriority=25  DisablePreemption=on  ClearInterruptFlagsAtEndOfEvent=on  InterruptDefinitionFile=$(TARGET_ROOT)/registry/interrupts/F2837xS_interrupts.xml  HardwareBoard=F2837x  EnableSimPort=off
      settings: LibrarySourceBlock=c2000lib/Scheduling/Hardware Interrupt
  HW_INT_ECAP2 : svdschedulerlib/Hardware Interrupt v2  ISRGroup=ADC - Analog to Digital Converter  ISRName=ADCA1_INT  ISRNumber=32  NumEventsToServe=1  EventsList={'on','EOC event','1';'off','Overflow event','2';'off','Custom event','3'}  SelectedEvents={'event1'}  TaskPriority=25  DisablePreemption=on  ClearInterruptFlagsAtEndOfEvent=on  InterruptDefinitionFile=$(TARGET_ROOT)/registry/interrupts/F2837xS_interrupts.xml  HardwareBoard=F2837x  EnableSimPort=off
      settings: LibrarySourceBlock=c2000lib/Scheduling/Hardware Interrupt
  HW_INT_ECAP3 : svdschedulerlib/Hardware Interrupt v2  ISRGroup=ADC - Analog to Digital Converter  ISRName=ADCA1_INT  ISRNumber=32  NumEventsToServe=1  EventsList={'on','EOC event','1';'off','Overflow event','2';'off','Custom event','3'}  SelectedEvents={'event1'}  TaskPriority=25  DisablePreemption=on  ClearInterruptFlagsAtEndOfEvent=on  InterruptDefinitionFile=$(TARGET_ROOT)/registry/interrupts/F2837xS_interrupts.xml  HardwareBoard=F2837x  EnableSimPort=off
      settings: LibrarySourceBlock=c2000lib/Scheduling/Hardware Interrupt
  Mux : Mux
  HW_INT : Outport
  wires:
  HW_INT_ECAP2/1 -> Mux/3
  HW_INT_ECAP1/1 -> Mux/2
  HW_INT_ECAP3/1 -> Mux/4
  HW_INT_ADCB1/1 -> Mux/1
  Mux/1 -> HW_INT/1

== system impmodel/Code Generation/Simulation ==
  Function-Call Generator{,1..3} (4 alike) : simulink/Ports & Subsystems/Function-Call Generator  sample_time=T_pwm  numberOfIterations=1  DisallowWideOutput=off
  Mux : Mux
  HW_INT : Outport
  wires:
  Mux/1 -> HW_INT/1
  Function-Call Generator/1 -> Mux/1
  Function-Call Generator1/1 -> Mux/2
  Function-Call Generator2/1 -> Mux/3
  Function-Call Generator3/1 -> Mux/4

== system impmodel/Hall Sensor A/Capture Event Selection ==
  Hall State : Inport
  If : If  IfExpression=(u1 == 5 | u1 == 3)
  Merge : Merge
  Output 0 : Subsystem  TreatAsAtomicUnit=on
  Output 1 : Subsystem  TreatAsAtomicUnit=on
  Capture Event Select : Outport
  wires:
  Hall State/1 -> If/1
  Merge/1 -> Capture Event Select/1
  Output 0/1(Out1) -> Merge/2
  If/2 -> Output 0/Action
  If/1 -> Output 1/Action
  Output 1/1(Out1) -> Merge/1

== system impmodel/Hall Sensor A/Code generation ==
  eCAP : c280xlib/eCAP  operatingMode=eCAP  selectCAPx=eCAP1  offsetValue=0  counterSynIn=off  enableCounter=off  syncOutput=Pass through  sampleTime=-1  eventPrescaler=0  selectMode=Continuous  enableOneShot=off  stopValue=Capture Event 2  resetEv1Ts=on  ev1Polarity=Rising Edge  resetEv2Ts=on  ev2Polarity=Falling Edge  resetEv3Ts=off  ev3Polarity=Rising Edge  resetEv4Ts=off  ev4Polarity=Rising Edge  tSCntrDataType=uint32  capEvFlag=off  capFlagDataType=uint32  overFlowFlag=off  overFlowFlagDataType=uint16  periodUnit=Seconds  periodSource=Specify via dialog  waveformPeriod=0.001  dutyUnit=Percentages  dutySource=Specify via dialog  dutyCycle=50  outputPolarity=Active High  enableCEVT1Int=on  enableCEVT2Int=on  enableCEVT3Int=off  enableCEVT4Int=off  enableCTROVFInt=on  enablePRDInt=off  enableCMPInt=off
      settings: LibrarySourceBlock=c2838xlib/eCAP
  eCAP_Out : Outport
  wires:
  eCAP/1 -> eCAP_Out/1

== system impmodel/Hall Sensor A/CodeGen ==
  Bitwise OR : simulink/Logic and Bit Operations/Bitwise Operator  logicop=OR  UseBitMask=off  NumInputPorts=3  BitMask=bin2dec('11011001')  BitMaskRealWorld=Stored Integer
      settings: LibrarySourceBlock=|
      | simulink/Quick Insert/Logic and Bit
      | Operations/Bitwise OR
  Data Store Write : DataStoreWrite  DataStoreName=HallC  IndexOptions=Index vector (dialog)  Indices=1  OutputSizes=1
  Data Store Write1 : DataStoreWrite  DataStoreName=HallB  IndexOptions=Index vector (dialog)  Indices=1  OutputSizes=1
  Data Store Write2 : DataStoreWrite  DataStoreName=HallA  IndexOptions=Index vector (dialog)  Indices=1  OutputSizes=1
  Data Type Conversion : DataTypeConversion  OutDataTypeStr=uint32  ConvertRealWorld=Stored Integer (SI)  SaturateOnIntegerOverflow=off  RndMeth=Floor
  GPIO 24 Hall_A : simulink/Logic and Bit Operations/Bitwise Operator  logicop=AND  UseBitMask=on  BitMask=hex2dec('1000000')  BitMaskRealWorld=Stored Integer
      settings: LibrarySourceBlock=|
      | simulink/Quick Insert/Logic and Bit
      | Operations/Bitwise AND
  GPIO 25 Hall_B : simulink/Logic and Bit Operations/Bitwise Operator  logicop=AND  UseBitMask=on  BitMask=hex2dec('2000000')  BitMaskRealWorld=Stored Integer
      settings: LibrarySourceBlock=|
      | simulink/Quick Insert/Logic and Bit
      | Operations/Bitwise AND
  GPIO 26 Hall_C : simulink/Logic and Bit Operations/Bitwise Operator  logicop=AND  UseBitMask=on  BitMask=hex2dec('4000000')  BitMaskRealWorld=Stored Integer
      settings: LibrarySourceBlock=|
      | simulink/Quick Insert/Logic and Bit
      | Operations/Bitwise AND
  Memory Copy : idelinklib_common/Memory Copy  copyFrom=Specified source code symbol  copyFromAddressSource=Specify via dialog  copyFromAddress=hex2dec('00001000')  copyFromSrcCode=&GpioDataRegs.GPADAT.all  dataTypeFrom=uint32  dataDimensionFrom=1  useOffsetFrom=off  offsetFromSrc=Specify via dialog  offsetFrom=0  strideFrom=1  copyTo=Output port  copyToAddressSource=Specify via dialog  copyToAddress=hex2dec('00002000')  copyToSrcCode=myVariableDst  dataTypeTo=uint32  useOffsetTo=off  offsetToSrc=Specify via dialog  offsetTo=0  strideTo=1  sampleTime=-1  useInitValue=off  initValueSrc=Specify constant value  initValue=1  initValueSrcCode=myInitValueVariable  useAsMask=off  maskOperator=bitwise AND  useTermValue=off  termValue=1  isRealtimeEnabled=off  emitCCBeforeWrite=off  CCBeforeWrite=/* Custom Code Before Write*/  emitCCAfterWrite=off  CCAfterWrite=/* Custom Code After Write*/
  Shift Arithmetic : ArithShift  BitShiftNumber=26
  Shift Arithmetic1 : ArithShift  BitShiftNumber=24
  Shift Arithmetic2 : ArithShift  BitShiftNumber=22
  Out1 : Outport
  wires:
  Data Type Conversion/1 -> Out1/1
  GPIO 26 Hall_C/1 -> Shift Arithmetic/1
  Bitwise OR/1 -> Data Type Conversion/1
  Shift Arithmetic/1 -> Data Store Write/1, Bitwise OR/1
  GPIO 24 Hall_A/1 -> Shift Arithmetic2/1
  Shift Arithmetic1/1 -> Data Store Write1/1, Bitwise OR/2
  Shift Arithmetic2/1 -> Data Store Write2/1, Bitwise OR/3
  Memory Copy/1 -> GPIO 25 Hall_B/1, GPIO 24 Hall_A/1, GPIO 26 Hall_C/1
  GPIO 25 Hall_B/1 -> Shift Arithmetic1/1

== system impmodel/Hall Sensor B/Capture Event Selection ==
  Hall State : Inport
  If : If  IfExpression=(u1 == 3 | u1 == 6)
  Merge : Merge
  Output 0 : Subsystem  TreatAsAtomicUnit=on
  Output 1 : Subsystem  TreatAsAtomicUnit=on
  Capture Event Select : Outport
  wires:
  Hall State/1 -> If/1
  Merge/1 -> Capture Event Select/1
  Output 0/1(Out1) -> Merge/2
  If/2 -> Output 0/Action
  If/1 -> Output 1/Action
  Output 1/1(Out1) -> Merge/1

== system impmodel/Hall Sensor B/Code generation ==
  eCAP : c280xlib/eCAP  operatingMode=eCAP  selectCAPx=eCAP2  offsetValue=0  counterSynIn=off  enableCounter=off  syncOutput=Pass through  sampleTime=-1  eventPrescaler=0  selectMode=Continuous  enableOneShot=off  stopValue=Capture Event 2  resetEv1Ts=on  ev1Polarity=Rising Edge  resetEv2Ts=on  ev2Polarity=Falling Edge  resetEv3Ts=off  ev3Polarity=Rising Edge  resetEv4Ts=off  ev4Polarity=Rising Edge  tSCntrDataType=uint32  capEvFlag=off  capFlagDataType=uint16  overFlowFlag=off  overFlowFlagDataType=uint16  periodUnit=Seconds  periodSource=Specify via dialog  waveformPeriod=0.001  dutyUnit=Percentages  dutySource=Specify via dialog  dutyCycle=50  outputPolarity=Active High  enableCEVT1Int=on  enableCEVT2Int=on  enableCEVT3Int=off  enableCEVT4Int=off  enableCTROVFInt=on  enablePRDInt=off  enableCMPInt=off
      settings: LibrarySourceBlock=c2838xlib/eCAP
  eCAP_Out : Outport
  wires:
  eCAP/1 -> eCAP_Out/1

== system impmodel/Hall Sensor B/CodeGen ==
  Bitwise OR : simulink/Logic and Bit Operations/Bitwise Operator  logicop=OR  UseBitMask=off  NumInputPorts=3  BitMask=bin2dec('11011001')  BitMaskRealWorld=Stored Integer
      settings: LibrarySourceBlock=|
      | simulink/Quick Insert/Logic and Bit
      | Operations/Bitwise OR
  Data Store Write : DataStoreWrite  DataStoreName=HallC  IndexOptions=Index vector (dialog)  Indices=1  OutputSizes=1
  Data Store Write1 : DataStoreWrite  DataStoreName=HallB  IndexOptions=Index vector (dialog)  Indices=1  OutputSizes=1
  Data Store Write2 : DataStoreWrite  DataStoreName=HallA  IndexOptions=Index vector (dialog)  Indices=1  OutputSizes=1
  Data Type Conversion : DataTypeConversion  OutDataTypeStr=uint32  ConvertRealWorld=Stored Integer (SI)  SaturateOnIntegerOverflow=off  RndMeth=Floor
  GPIO 24 Hall_A : simulink/Logic and Bit Operations/Bitwise Operator  logicop=AND  UseBitMask=on  BitMask=hex2dec('1000000')  BitMaskRealWorld=Stored Integer
      settings: LibrarySourceBlock=|
      | simulink/Quick Insert/Logic and Bit
      | Operations/Bitwise AND
  GPIO 25 Hall_B : simulink/Logic and Bit Operations/Bitwise Operator  logicop=AND  UseBitMask=on  BitMask=hex2dec('2000000')  BitMaskRealWorld=Stored Integer
      settings: LibrarySourceBlock=|
      | simulink/Quick Insert/Logic and Bit
      | Operations/Bitwise AND
  GPIO 26 Hall_C : simulink/Logic and Bit Operations/Bitwise Operator  logicop=AND  UseBitMask=on  BitMask=hex2dec('4000000')  BitMaskRealWorld=Stored Integer
      settings: LibrarySourceBlock=|
      | simulink/Quick Insert/Logic and Bit
      | Operations/Bitwise AND
  Memory Copy : idelinklib_common/Memory Copy  copyFrom=Specified source code symbol  copyFromAddressSource=Specify via dialog  copyFromAddress=hex2dec('00001000')  copyFromSrcCode=&GpioDataRegs.GPADAT.all  dataTypeFrom=uint32  dataDimensionFrom=1  useOffsetFrom=off  offsetFromSrc=Specify via dialog  offsetFrom=0  strideFrom=1  copyTo=Output port  copyToAddressSource=Specify via dialog  copyToAddress=hex2dec('00002000')  copyToSrcCode=myVariableDst  dataTypeTo=uint32  useOffsetTo=off  offsetToSrc=Specify via dialog  offsetTo=0  strideTo=1  sampleTime=-1  useInitValue=off  initValueSrc=Specify constant value  initValue=1  initValueSrcCode=myInitValueVariable  useAsMask=off  maskOperator=bitwise AND  useTermValue=off  termValue=1  isRealtimeEnabled=off  emitCCBeforeWrite=off  CCBeforeWrite=/* Custom Code Before Write*/  emitCCAfterWrite=off  CCAfterWrite=/* Custom Code After Write*/
  Shift Arithmetic : ArithShift  BitShiftNumber=26
  Shift Arithmetic1 : ArithShift  BitShiftNumber=24
  Shift Arithmetic2 : ArithShift  BitShiftNumber=22
  Out1 : Outport
  wires:
  Data Type Conversion/1 -> Out1/1
  Shift Arithmetic2/1 -> Data Store Write2/1, Bitwise OR/3
  Shift Arithmetic1/1 -> Data Store Write1/1, Bitwise OR/2
  Memory Copy/1 -> GPIO 26 Hall_C/1, GPIO 25 Hall_B/1, GPIO 24 Hall_A/1
  Shift Arithmetic/1 -> Data Store Write/1, Bitwise OR/1
  Bitwise OR/1 -> Data Type Conversion/1
  GPIO 24 Hall_A/1 -> Shift Arithmetic2/1
  GPIO 25 Hall_B/1 -> Shift Arithmetic1/1
  GPIO 26 Hall_C/1 -> Shift Arithmetic/1

== system impmodel/Hall Sensor C/Capture Event Selection ==
  Hall State : Inport
  If : If  IfExpression=(u1 == 5 | u1 == 6)
  Merge : Merge
  Output 0 : Subsystem  TreatAsAtomicUnit=on
  Output 1 : Subsystem  TreatAsAtomicUnit=on
  Capture Event Select : Outport
  wires:
  Hall State/1 -> If/1
  Merge/1 -> Capture Event Select/1
  Output 0/1(Out1) -> Merge/2
  If/2 -> Output 0/Action
  If/1 -> Output 1/Action
  Output 1/1(Out1) -> Merge/1

== system impmodel/Hall Sensor C/Code generation ==
  eCAP : c280xlib/eCAP  operatingMode=eCAP  selectCAPx=eCAP3  offsetValue=0  counterSynIn=off  enableCounter=off  syncOutput=Disabled  sampleTime=-1  eventPrescaler=0  selectMode=Continuous  enableOneShot=off  stopValue=Capture Event 2  resetEv1Ts=on  ev1Polarity=Rising Edge  resetEv2Ts=on  ev2Polarity=Falling Edge  resetEv3Ts=off  ev3Polarity=Rising Edge  resetEv4Ts=off  ev4Polarity=Rising Edge  tSCntrDataType=uint32  capEvFlag=off  capFlagDataType=uint16  overFlowFlag=off  overFlowFlagDataType=uint16  periodUnit=Seconds  periodSource=Specify via dialog  waveformPeriod=0.001  dutyUnit=Percentages  dutySource=Specify via dialog  dutyCycle=50  outputPolarity=Active High  enableCEVT1Int=on  enableCEVT2Int=on  enableCEVT3Int=off  enableCEVT4Int=off  enableCTROVFInt=on  enablePRDInt=off  enableCMPInt=off
      settings: LibrarySourceBlock=c2838xlib/eCAP
  eCAP_Out : Outport
  wires:
  eCAP/1 -> eCAP_Out/1

== system impmodel/Hall Sensor C/CodeGen ==
  Bitwise OR : simulink/Logic and Bit Operations/Bitwise Operator  logicop=OR  UseBitMask=off  NumInputPorts=3  BitMask=bin2dec('11011001')  BitMaskRealWorld=Stored Integer
      settings: LibrarySourceBlock=|
      | simulink/Quick Insert/Logic and Bit
      | Operations/Bitwise OR
  Data Store Write : DataStoreWrite  DataStoreName=HallC  IndexOptions=Index vector (dialog)  Indices=1  OutputSizes=1
  Data Store Write1 : DataStoreWrite  DataStoreName=HallB  IndexOptions=Index vector (dialog)  Indices=1  OutputSizes=1
  Data Store Write2 : DataStoreWrite  DataStoreName=HallA  IndexOptions=Index vector (dialog)  Indices=1  OutputSizes=1
  Data Type Conversion : DataTypeConversion  OutDataTypeStr=uint32  ConvertRealWorld=Stored Integer (SI)  SaturateOnIntegerOverflow=off  RndMeth=Floor
  GPIO 24 Hall_A : simulink/Logic and Bit Operations/Bitwise Operator  logicop=AND  UseBitMask=on  BitMask=hex2dec('1000000')  BitMaskRealWorld=Stored Integer
      settings: LibrarySourceBlock=|
      | simulink/Quick Insert/Logic and Bit
      | Operations/Bitwise AND
  GPIO 25 Hall_B : simulink/Logic and Bit Operations/Bitwise Operator  logicop=AND  UseBitMask=on  BitMask=hex2dec('2000000')  BitMaskRealWorld=Stored Integer
      settings: LibrarySourceBlock=|
      | simulink/Quick Insert/Logic and Bit
      | Operations/Bitwise AND
  GPIO 26 Hall_C : simulink/Logic and Bit Operations/Bitwise Operator  logicop=AND  UseBitMask=on  BitMask=hex2dec('4000000')  BitMaskRealWorld=Stored Integer
      settings: LibrarySourceBlock=|
      | simulink/Quick Insert/Logic and Bit
      | Operations/Bitwise AND
  Memory Copy : idelinklib_common/Memory Copy  copyFrom=Specified source code symbol  copyFromAddressSource=Specify via dialog  copyFromAddress=hex2dec('00001000')  copyFromSrcCode=&GpioDataRegs.GPADAT.all  dataTypeFrom=uint32  dataDimensionFrom=1  useOffsetFrom=off  offsetFromSrc=Specify via dialog  offsetFrom=0  strideFrom=1  copyTo=Output port  copyToAddressSource=Specify via dialog  copyToAddress=hex2dec('00002000')  copyToSrcCode=myVariableDst  dataTypeTo=uint32  useOffsetTo=off  offsetToSrc=Specify via dialog  offsetTo=0  strideTo=1  sampleTime=-1  useInitValue=off  initValueSrc=Specify constant value  initValue=1  initValueSrcCode=myInitValueVariable  useAsMask=off  maskOperator=bitwise AND  useTermValue=off  termValue=1  isRealtimeEnabled=off  emitCCBeforeWrite=off  CCBeforeWrite=/* Custom Code Before Write*/  emitCCAfterWrite=off  CCAfterWrite=/* Custom Code After Write*/
  Shift Arithmetic : ArithShift  BitShiftNumber=26
  Shift Arithmetic1 : ArithShift  BitShiftNumber=24
  Shift Arithmetic2 : ArithShift  BitShiftNumber=22
  Out1 : Outport
  wires:
  Data Type Conversion/1 -> Out1/1
  Shift Arithmetic2/1 -> Data Store Write2/1, Bitwise OR/3
  Shift Arithmetic1/1 -> Data Store Write1/1, Bitwise OR/2
  Memory Copy/1 -> GPIO 26 Hall_C/1, GPIO 25 Hall_B/1, GPIO 24 Hall_A/1
  Shift Arithmetic/1 -> Data Store Write/1, Bitwise OR/1
  Bitwise OR/1 -> Data Type Conversion/1
  GPIO 24 Hall_A/1 -> Shift Arithmetic2/1
  GPIO 25 Hall_B/1 -> Shift Arithmetic1/1
  GPIO 26 Hall_C/1 -> Shift Arithmetic/1

== system impmodel/IPC Write for eCAP INTs/TCP_HallA ==
  " " : Inport
  Data_Type_Fixed_Point : Subsystem  VariantControl=~isequal(dataType,'single')
  Interprocess Data Write : procinterlib/Interprocess Data Write  showPort=off  ChannelNum=3  NumBuff=1  IsIntEnabled=1  EnInterrupt=on  IPCBetween=1  CurrentPU=0  DataType=uint8  PartCores=CPU1<->CM  TargetType=0  ClientPU=TriCore1  ClientIntPrio=50
  wires:
  Data_Type_Fixed_Point/1(Data_Log) -> Interprocess Data Write/1
  " "/1 -> Data_Type_Fixed_Point/1(In1)

== system impmodel/IPC Write for eCAP INTs/TCP_HallB ==
  " " : Inport
  Data_Type_Fixed_Point : Subsystem  VariantControl=~isequal(dataType,'single')
  Interprocess Data Write : procinterlib/Interprocess Data Write  showPort=off  ChannelNum=4  NumBuff=1  IsIntEnabled=1  EnInterrupt=on  IPCBetween=1  CurrentPU=0  DataType=uint8  PartCores=CPU1<->CM  TargetType=0  ClientPU=TriCore1  ClientIntPrio=50
  wires:
  " "/1 -> Data_Type_Fixed_Point/1(In1)
  Data_Type_Fixed_Point/1(Data_Log) -> Interprocess Data Write/1

== system impmodel/IPC Write for eCAP INTs/TCP_HallC ==
  " " : Inport
  Data_Type_Fixed_Point : Subsystem  VariantControl=~isequal(dataType,'single')
  Interprocess Data Write : procinterlib/Interprocess Data Write  showPort=off  ChannelNum=5  NumBuff=1  IsIntEnabled=1  EnInterrupt=on  IPCBetween=1  CurrentPU=0  DataType=uint8  PartCores=CPU1<->CM  TargetType=0  ClientPU=TriCore1  ClientIntPrio=50
  wires:
  Data_Type_Fixed_Point/1(Data_Log) -> Interprocess Data Write/1
  " "/1 -> Data_Type_Fixed_Point/1(In1)

== system impmodel/IPC Write for eCAP INTs/TCP_HallState ==
  " " : Inport
  Data_Type_Fixed_Point : Subsystem  VariantControl=~isequal(dataType,'single')
  Interprocess Data Write : procinterlib/Interprocess Data Write  showPort=off  ChannelNum=2  NumBuff=1  IsIntEnabled=1  EnInterrupt=on  IPCBetween=1  CurrentPU=0  DataType=uint8  PartCores=CPU1<->CM  TargetType=0  ClientPU=TriCore1  ClientIntPrio=50
  wires:
  " "/1 -> Data_Type_Fixed_Point/1(In1)
  Data_Type_Fixed_Point/1(Data_Log) -> Interprocess Data Write/1

== system impmodel/Input Controller/BatteryVoltage_CodeGen ==
  " " : c2802xlib/ADC  blkParamProc=C2000_Type4  ADCModule=A  samplingMode=Single sample mode  ADCResolution=12-bit (Single-ended input)  useSOC1=SOC3  useSOC2=SOC0_SOC1  SOCAcquisitionWindow=8  SOCTriggerSource=Software  SOCInterruptTrigger=No ADCINT  Ts=0.2  dType=uint16  postInterrupt=off  interruptSel=ADCINT1  ADCINTContinuous=on  endma=off  chdma=1  conv1=ADCINA0  conv2=ADCINA0 and ADCINB0  conv1_Type4=ADCIN5  conv2_Type4=ADCIN0 and ADCIN1
      settings: LibrarySourceBlock=c2838xlib/ADC
  Data Type Conversion : DataTypeConversion  OutDataTypeStr=single  SaturateOnIntegerOverflow=off  RndMeth=Floor
  Data Type Conversion1 : DataTypeConversion  OutDataTypeStr=uint16  RndMeth=Nearest  SaturateOnIntegerOverflow=off
  Divide : Product  Inputs=*/  OutDataTypeStr=Inherit: Same as first input
  Product : Product  OutDataTypeStr=Inherit: Same as first input
  Product2 : Product  OutDataTypeStr=Inherit: Same as first input
  R1+R2 : Constant  Value=100610  OutDataTypeStr=single  SampleTime=-1
  R2 : Constant  Value=3010  OutDataTypeStr=single  SampleTime=-1
  Scaling : Constant  Value=target_f2838.ADC_Vref/target_f2838.ADC_MaxCount  OutDataTypeStr=single  SampleTime=-1
  eCAN Transmit : c280xlib/eCAN Transmit  chipFamily=C280x  useModule=eCAN_A  mailboxNo=1  messageID=hex2dec('110')  messageType=Standard (11-bit identifier)  enableBlockingMode=off  postInterrupt=off  interruptLine=0
      settings: LibrarySourceBlock=c28004xlib/eCAN Transmit
  batteryVoltage : Outport
  wires:
  Data Type Conversion/1 -> Product/1
  Product/1 -> Divide/1
  Scaling/1 -> Product/2
  R2/1 -> Divide/2
  Divide/1 -> Product2/1
  R1+R2/1 -> Product2/2
  Product2/1 -> Data Type Conversion1/1
  Data Type Conversion1/1 -> batteryVoltage/1, eCAN Transmit/1
  " "/1 -> Data Type Conversion/1

== system impmodel/Input Controller/Freemode_Sig_CodeGen ==
  Data Type Conversion : DataTypeConversion  OutDataTypeStr=fixdt(1,32,17)  SaturateOnIntegerOverflow=off  RndMeth=Floor
  Saturation : Saturate  UpperLimit=1  LowerLimit=0
  Select first element : Selector  InputPortWidth=4  IndexOptions=Index vector (dialog)  Indices=[1]  OutputSizes=1
  Terminator : Terminator
  eCAN Receive : c280xlib/eCAN Receive  chipFamily=C280x  useModule=eCAN_A  mailboxNo=9  messageID=hex2dec('101')  messageType=Standard (11-bit identifier)  enableAcceptanceFiltering=off  messageIDMask=0  sampleTime=0.2  dataType=uint16  outputAction=Output last received values  initValue=0  outputMessageID=off  outputMessageLength=off  outputMessageTimeStamp=off  postInterrupt=off  interruptLine=0
      settings: LibrarySourceBlock=c28004xlib/eCAN Receive
  Freemode_Sig : Outport
  wires:
  eCAN Receive/1 -> Terminator/1
  eCAN Receive/2 -> Select first element/1
  Data Type Conversion/1 -> Saturation/1
  Select first element/1 -> Data Type Conversion/1
  Saturation/1 -> Freemode_Sig/1

== system impmodel/Input Controller/GVDD_Calculation ==
  ADC : c2802xlib/ADC  blkParamProc=C2000_Type5  ADCModule=C  samplingMode=Single sample mode  ADCResolution=12-bit (Single-ended input)  useSOC1=SOC4  useSOC2=SOC0_SOC1  SOCAcquisitionWindow=8  SOCTriggerSource=Software  SOCInterruptTrigger=No ADCINT  Ts=0.2  dType=uint16  postInterrupt=off  interruptSel=ADCINT1  ADCINTContinuous=on  endma=off  chdma=1  conv1=ADCINA0  conv2=ADCINA0 and ADCINB0  conv1_Type4=ADCIN3  conv2_Type4=ADCIN0 and ADCIN1
      settings: LibrarySourceBlock=c28004xlib/ADC
  Data Type Conversion : DataTypeConversion  OutDataTypeStr=single  SaturateOnIntegerOverflow=off  RndMeth=Floor
  Data Type Conversion1 : DataTypeConversion  OutDataTypeStr=uint16  RndMeth=Nearest  SaturateOnIntegerOverflow=off
  Divide : Product  Inputs=*/  OutDataTypeStr=Inherit: Same as first input
  Product : Product  OutDataTypeStr=Inherit: Same as first input
  Product2 : Product  OutDataTypeStr=Inherit: Same as first input
  R1+R2 : Constant  Value=100610  OutDataTypeStr=single  SampleTime=-1
  R2 : Constant  Value=3010  OutDataTypeStr=single  SampleTime=-1
  Scaling : Constant  Value=target_f2838.ADC_Vref/target_f2838.ADC_MaxCount  OutDataTypeStr=single  SampleTime=-1
  eCAN Transmit : c280xlib/eCAN Transmit  chipFamily=C280x  useModule=eCAN_A  mailboxNo=1  messageID=hex2dec('111')  messageType=Standard (11-bit identifier)  enableBlockingMode=off  postInterrupt=off  interruptLine=0
      settings: LibrarySourceBlock=c28004xlib/eCAN Transmit
  wires:
  Data Type Conversion1/1 -> eCAN Transmit/1
  Product2/1 -> Data Type Conversion1/1
  R1+R2/1 -> Product2/2
  Divide/1 -> Product2/1
  R2/1 -> Divide/2
  Scaling/1 -> Product/2
  Product/1 -> Divide/1
  Data Type Conversion/1 -> Product/1
  ADC/1 -> Data Type Conversion/1

== system impmodel/Input Controller/SafeState_CodeGen ==
  SafeState_Pin : c2838xlib/Digital Input  GPIO_Number=GPIO24~GPIO31  GPIO_Bit0=off  GPIO_Bit1=off  GPIO_Bit2=off  GPIO_Bit3=off  GPIO_Bit4=off  GPIO_Bit5=off  GPIO_Bit6=on  GPIO_Bit7=off  sampleTime=0.2  dataType=boolean  GPIO_Bit0_Qualification=Sync to SYSCLKOUT  GPIO_Bit1_Qualification=Sync to SYSCLKOUT  GPIO_Bit2_Qualification=Sync to SYSCLKOUT  GPIO_Bit3_Qualification=Sync to SYSCLKOUT  GPIO_Bit4_Qualification=Sync to SYSCLKOUT  GPIO_Bit5_Qualification=Sync to SYSCLKOUT  GPIO_Bit6_Qualification=Sync to SYSCLKOUT  GPIO_Bit7_Qualification=Sync to SYSCLKOUT  Qualification_Period=-1
  SafeState_CodeGen : Outport
  wires:
  SafeState_Pin/1 -> SafeState_CodeGen/1

== system impmodel/Input Controller/Speed Command_Sim ==
  Data Type Conversion : DataTypeConversion  OutDataTypeStr=fixdt(1,32,17)  SaturateOnIntegerOverflow=off  RndMeth=Floor
  Reversal : Step  Commented=on  Time=5  SampleTime=0.01
  Sine Wave : Sin  Commented=on  Amplitude=0.9  Frequency=0.2  SampleTime=0.01
  Speed_Ref_Final (rpm) : Constant  Commented=on  Value=0  OutDataTypeStr=double  SampleTime=0.01
  Step : Step  After=0.25  SampleTime=0.01
  Switch : Switch  Commented=on  Criteria=u2 > Threshold  SaturateOnIntegerOverflow=off  InputSameDT=off
  Speed_Ref : Outport
  wires:
  Reversal/1 -> Switch/2
  Sine Wave/1 -> Switch/3
  Speed_Ref_Final (rpm)/1 -> Switch/1
  Data Type Conversion/1 -> Speed_Ref/1
  Step/1 -> Data Type Conversion/1
